simulink model "IEEE_BUS_68_AGC"  (R2025a)
settings: Solver=ode23tb  StartTime=0.0  StopTime=150  FixedStep=Ts  MaxStep=0.0001  RelTol=1e-3
PreLoadFcn:
  | PSSMODEL=1;
  | LPSS=0;
  | WAPSS=0;
  | WAPSS2=0;
  | Ts=50e-5;
InitFcn:
  | PSSMODEL=1;
  | LPSS=0;
  | WAPSS=0;
  | WAPSS2=0;
  | Ts=50e-5;
  | 
  | % Required data to 68 Bus benchmark
  | % clear
  | % clc
  | % Definition for the columns
  | % system base =100 MVA
  | 
  | %% Line data Format (line)
  | % All values are given on the same system base MVA
  | % 1: From bus
  | % 2: To bus
  | % 3: Resistance (pu)
  | % 4: Reactance  (pu)
  | % 5: Charge     (pu)
  | % 6: Transformer Tap Amplitute
  | % 7: base MVA
  | % 8: Nomonal Voltage (KV)
  | 
  | %1   2    3        4       5       6        7      8
  | line=[...
  | 1	54	0	     0.0181	  0	      1.025     100    13.8
  | 2	58	0	     0.025	  0	      1.070     100    13.8
  | 3	62	0	     0.02	  0	      1.070     100    13.8
  | 4	19	0.0007	 0.0142	  0	      1.070     100    13.8
  | 5	20	0.0009	 0.018	  0	      1.009     100    13.8
  | 6	22	0	     0.0143	  0	      1.025     100    13.8
  | 7	23	0.0005	 0.0272	  0	      0         100    13.8
  | 8	25	0.0006	 0.0232	  0	      1.025     100    13.8
  | 9	29	0.0008	 0.0156   0	      1.025     100    13.8
  | 10	31	0	     0.026	  0	      1.04      100    13.8
  | 11	32	0	     0.013	  0	      1.04      100    13.8
  | 12	36	0	     0.0075	  0	      1.04      100    13.8
  | 13	17	0	     0.0033	  0	      1.04      100    13.8
  | 14	41	0	     0.0015	  0	      1         100    13.8
  | 15	42	0	     0.0015	  0	      1         100    13.8
  | 16	18	0	     0.003	  0	      1         100    13.8
  | 17	36	0.0005	 0.0045	  0.32	  0         100    138
  | 17	43	0.0005	 0.0276	  0	      0         100    138
  | 18	42	0.004	 0.06	  2.25    0         100    138
  | 18	49	0.0076	 0.1141	  1.16    0	        100    138
  | 18	50	0.0012	 0.0288	  2.06	  0         100    138
  | 20	19	0.0007	 0.0138	  0       1.06	    100    138
  | 19	68	0.0016	 0.0195	  0.304	  0         100    138
  | 21	22	0.0008	 0.014	  0.2565  0	        100    138
  | 21	68	0.0008	 0.0135	  0.2548  0	        100    138
  | 22	23	0.0006	 0.0096	  0.1846  0	        100    138
  | 23	24	0.0022	 0.035	  0.361	  0         100    138
  | 24	68	0.0003	 0.0059	  0.068	  0         100    138
  | 25	26	0.0032	 0.0323	  0.531	  0         100    138
  | 25	54	0.007	 0.0086	  0.146	  0         100    138
  | 26	27	0.0014	 0.0147	  0.2396  0	        100    138
  | 26	28	0.0043	 0.0474	  0.7802  0	        100    138
  | 26	29	0.0057	 0.0625	  1.029	  0         100    138
  | 27	37	0.0013	 0.0173	  0.3216  0	        100    138
  | 27	53	0.032	 0.32	  0.41	  0         100    138
  | ... (+206 lines)
undefined symbols (not defined in the file or in its folder): D1, Delta
libraries: spsPMUPLLBasedPositiveSequenceLib x90, spsRMSLib x73, spsThreePhaseVIMeasurementLib x69, spsLoadFlowBusLib x69, spsThreePhasePISectionLineLib x64, spsThreePhaseParallelRLCLoadLib x35, spsGenericPowerSystemStabilizerLib x32, spsThreePhaseSeriesRLCLoadLib x21, spsThreePhaseTransformerTwoWindingsLib x21, spsSynchronousMachinepuStandardLib x20, spsExcitationSystemLib x16, spsMultiBandPowerSystemStabilizerLib x16
(part 3 of 8)

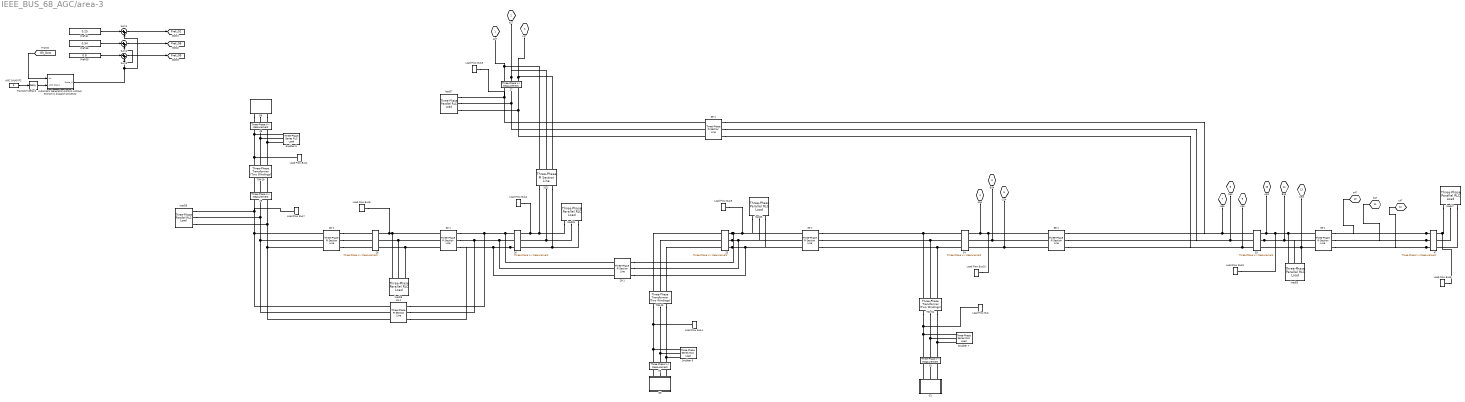
== system IEEE_BUS_68_AGC/area-3 ==
  01 : spsThreePhaseVIMeasurementLib/Three-Phase V-I Measurement  VoltageMeasurement=phase-to-phase  SetLabelV=on  LabelV=Vabc_01  Vpu=off  VpuLL=on  CurrentMeasurement=no  SetLabelI=off  LabelI=Iabc  Ipu=off  Pbase=100e6  Vbase=13.8e3  OutputType=Complex  PhasorSimulation=off  PSBequivalent=0
  08 : spsThreePhaseVIMeasurementLib/Three-Phase V-I Measurement  VoltageMeasurement=phase-to-phase  SetLabelV=on  LabelV=Vabc_08  Vpu=off  VpuLL=on  CurrentMeasurement=no  SetLabelI=off  LabelI=Iabc  Ipu=off  Pbase=100e6  Vbase=13.8e3  OutputType=Complex  PhasorSimulation=off  PSBequivalent=0
  09 : spsThreePhaseVIMeasurementLib/Three-Phase V-I Measurement  VoltageMeasurement=phase-to-phase  SetLabelV=on  LabelV=Vabc_09  Vpu=off  VpuLL=on  CurrentMeasurement=no  SetLabelI=off  LabelI=Iabc  Ipu=off  Pbase=100e6  Vbase=13.8e3  OutputType=Complex  PhasorSimulation=off  PSBequivalent=0
  25 : spsThreePhaseVIMeasurementLib/Three-Phase V-I Measurement  VoltageMeasurement=phase-to-phase  SetLabelV=on  LabelV=Vabc_25  Vpu=off  VpuLL=on  CurrentMeasurement=no  SetLabelI=off  LabelI=Iabc  Ipu=off  Pbase=100e6  Vbase=Bus(25,2)*1e3  OutputType=Complex  PhasorSimulation=off  PSBequivalent=0
  26 : spsThreePhaseVIMeasurementLib/Three-Phase V-I Measurement  VoltageMeasurement=phase-to-phase  SetLabelV=on  LabelV=Vabc_26  Vpu=off  VpuLL=on  CurrentMeasurement=no  SetLabelI=off  LabelI=Iabc  Ipu=off  Pbase=100e6  Vbase=Bus(26,2)*1e3  OutputType=Complex  PhasorSimulation=off  PSBequivalent=0
  27 : spsThreePhaseVIMeasurementLib/Three-Phase V-I Measurement  VoltageMeasurement=phase-to-phase  SetLabelV=on  LabelV=Vabc_27  Vpu=off  VpuLL=on  CurrentMeasurement=no  SetLabelI=off  LabelI=Iabc  Ipu=off  Pbase=100e6  Vbase=Bus(27,2)*1e3  OutputType=Complex  PhasorSimulation=off  PSBequivalent=0
  28 : spsThreePhaseVIMeasurementLib/Three-Phase V-I Measurement  VoltageMeasurement=phase-to-phase  SetLabelV=on  LabelV=Vabc_28  Vpu=off  VpuLL=on  CurrentMeasurement=no  SetLabelI=off  LabelI=Iabc  Ipu=off  Pbase=100e6  Vbase=Bus(28,2)*1e3  OutputType=Complex  PhasorSimulation=off  PSBequivalent=0
  29 : spsThreePhaseVIMeasurementLib/Three-Phase V-I Measurement  VoltageMeasurement=phase-to-phase  SetLabelV=on  LabelV=Vabc_29  Vpu=off  VpuLL=on  CurrentMeasurement=no  SetLabelI=off  LabelI=Iabc  Ipu=off  Pbase=100e6  Vbase=Bus(29,2)*1e3  OutputType=Complex  PhasorSimulation=off  PSBequivalent=0
  29-1 : spsThreePhasePISectionLineLib/Three-Phase PI Section Line  LConnTagsString=a|b|c  RConnTagsString=A|B|C  Length=1  Frequency=60  Resistances=[line(29,3) 3*line(29,3)]  Inductances=[line(29,4) 3*line(29,4)]  Capacitances=[line(29,5) line(29,5)/3]
  30-1 : spsThreePhasePISectionLineLib/Three-Phase PI Section Line  LConnTagsString=a|b|c  RConnTagsString=A|B|C  Length=1  Frequency=60  Resistances=[line(30,3) 3*line(30,3)]  Inductances=[line(30,4) 3*line(30,4)]  Capacitances=[line(30,5) line(30,5)/3]
  31-1 : spsThreePhasePISectionLineLib/Three-Phase PI Section Line  LConnTagsString=a|b|c  RConnTagsString=A|B|C  Length=1  Frequency=60  Resistances=[line(31,3) 3*line(31,3)]  Inductances=[line(31,4) 3*line(31,4)]  Capacitances=[line(31,5) line(31,5)/3]
  32-1 : spsThreePhasePISectionLineLib/Three-Phase PI Section Line  LConnTagsString=a|b|c  RConnTagsString=A|B|C  Length=1  Frequency=60  Resistances=[line(32,3) 3*line(32,3)]  Inductances=[line(32,4) 3*line(32,4)]  Capacitances=[line(32,5) line(32,5)/3]
  33-1 : spsThreePhasePISectionLineLib/Three-Phase PI Section Line  LConnTagsString=a|b|c  RConnTagsString=A|B|C  Length=1  Frequency=60  Resistances=[line(33,3) 3*line(33,3)]  Inductances=[line(33,4) 3*line(33,4)]  Capacitances=[line(33,5) line(33,5)/3]
  35-1 : spsThreePhasePISectionLineLib/Three-Phase PI Section Line  LConnTagsString=a|b|c  RConnTagsString=A|B|C  Length=1  Frequency=60  Resistances=[line(35,3) 3*line(35,3)]  Inductances=[line(35,4) 3*line(35,4)]  Capacitances=[line(35,5) line(35,5)/3]
  36-1 : spsThreePhasePISectionLineLib/Three-Phase PI Section Line  LConnTagsString=a|b|c  RConnTagsString=A|B|C  Length=1  Frequency=60  Resistances=[line(36,3) 3*line(36,3)]  Inductances=[line(36,4) 3*line(36,4)]  Capacitances=[line(36,5) line(36,5)/3]
  47 : spsThreePhaseVIMeasurementLib/Three-Phase V-I Measurement  VoltageMeasurement=phase-to-phase  SetLabelV=on  LabelV=Vabc_47  Vpu=off  VpuLL=on  CurrentMeasurement=no  SetLabelI=off  LabelI=Iabc  Ipu=off  Pbase=100e6  Vbase=Bus(47,2)*1e3  OutputType=Complex  PhasorSimulation=off  PSBequivalent=0
  53 : spsThreePhaseVIMeasurementLib/Three-Phase V-I Measurement  VoltageMeasurement=phase-to-phase  SetLabelV=on  LabelV=Vabc_53  Vpu=off  VpuLL=on  CurrentMeasurement=no  SetLabelI=off  LabelI=Iabc  Ipu=off  Pbase=100e6  Vbase=Bus(53,2)*1e3  OutputType=Complex  PhasorSimulation=off  PSBequivalent=0
  54 : spsThreePhaseVIMeasurementLib/Three-Phase V-I Measurement  VoltageMeasurement=phase-to-phase  SetLabelV=on  LabelV=Vabc_54  Vpu=off  VpuLL=on  CurrentMeasurement=no  SetLabelI=off  LabelI=Iabc  Ipu=off  Pbase=100e6  Vbase=Bus(54,2)*1e3  OutputType=Complex  PhasorSimulation=off  PSBequivalent=0
  63-1 : spsThreePhasePISectionLineLib/Three-Phase PI Section Line  LConnTagsString=a|b|c  RConnTagsString=A|B|C  Length=1  Frequency=60  Resistances=[line(63,3) 3*line(63,3)]  Inductances=[line(63,4) 3*line(63,4)]  Capacitances=[line(63,5) line(63,5)/3]
  66-1 : spsThreePhasePISectionLineLib/Three-Phase PI Section Line  LConnTagsString=a|b|c  RConnTagsString=A|B|C  Length=1  Frequency=60  Resistances=[line(66,3) 3*line(66,3)]  Inductances=[line(66,4) 3*line(66,4)]  Capacitances=[line(66,5) line(66,5)/3]
  AGC ON/OFF2 : Constant
  Automatic Generation Control without economic dispatch process2 : Subsystem
  G1 : Subsystem
  G8 : Subsystem
  G9 : Subsystem
  Load Flow Bus : spsLoadFlowBusLib/Load Flow Bus  LConnTagsString=a  Phases=single  Connectors=on one side  ID=BUS_01  Vbase=13.8e3  Vref=1.045  Vangle=0  VLF=1.045  VLFb=1  VLFc=1  angleLF=-12.3  angleLFb=0  angleLFc=0
  Load Flow Bus1 : spsLoadFlowBusLib/Load Flow Bus  LConnTagsString=a  Phases=single  Connectors=on one side  ID=BUS_09  Vbase=13.8e3  Vref=1.025  Vangle=0  VLF=1.025  VLFb=1  VLFc=1  angleLF=-5.821  angleLFb=0  angleLFc=0
  Load Flow Bus10 : spsLoadFlowBusLib/Load Flow Bus  LConnTagsString=a  Phases=single  Connectors=on one side  ID=BUS_54  Vbase=138e3  Vref=1  Vangle=0  VLF=1.017  VLFb=1  VLFc=1  angleLF=15.31  angleLFb=0  angleLFc=0
  Load Flow Bus2 : spsLoadFlowBusLib/Load Flow Bus  LConnTagsString=a  Phases=single  Connectors=on one side  ID=BUS_26  Vbase=138e3  Vref=1  Vangle=0  VLF=1.035  VLFb=1  VLFc=1  angleLF=15.99  angleLFb=0  angleLFc=0
  Load Flow Bus3 : spsLoadFlowBusLib/Load Flow Bus  LConnTagsString=a  Phases=single  Connectors=on one side  ID=BUS_27  Vbase=138e3  Vref=1  Vangle=0  VLF=1.025  VLFb=1  VLFc=1  angleLF=15.59  angleLFb=0  angleLFc=0
  Load Flow Bus4 : spsLoadFlowBusLib/Load Flow Bus  LConnTagsString=a  Phases=single  Connectors=on one side  ID=BUS_08  Vbase=13.8e3  Vref=1.03  Vangle=0  VLF=1.03  VLFb=1  VLFc=1  angleLF=-6.494  angleLFb=0  angleLFc=0
  Load Flow Bus5 : spsLoadFlowBusLib/Load Flow Bus  LConnTagsString=a  Phases=single  Connectors=on one side  ID=BUS_25  Vbase=138e3  Vref=1  Vangle=0  VLF=1.031  VLFb=1  VLFc=1  angleLF=16.75  angleLFb=0  angleLFc=0
  Load Flow Bus6 : spsLoadFlowBusLib/Load Flow Bus  LConnTagsString=a  Phases=single  Connectors=on one side  ID=BUS_28  Vbase=138e3  Vref=1  Vangle=0  VLF=1.028  VLFb=1  VLFc=1  angleLF=16.68  angleLFb=0  angleLFc=0
  Load Flow Bus7 : spsLoadFlowBusLib/Load Flow Bus  LConnTagsString=a  Phases=single  Connectors=on one side  ID=BUS_29  Vbase=138e3  Vref=1  Vangle=0  VLF=1.02  VLFb=1  VLFc=1  angleLF=17.35  angleLFb=0  angleLFc=0
  Load Flow Bus8 : spsLoadFlowBusLib/Load Flow Bus  LConnTagsString=a  Phases=single  Connectors=on one side  ID=BUS_47  Vbase=138e3  Vref=1  Vangle=0  VLF=1.027  VLFb=1  VLFc=1  angleLF=6.526  angleLFb=0  angleLFc=0
  Load Flow Bus9 : spsLoadFlowBusLib/Load Flow Bus  LConnTagsString=a  Phases=single  Connectors=on one side  ID=BUS_53  Vbase=138e3  Vref=1  Vangle=0  VLF=1.01  VLFb=1  VLFc=1  angleLF=8.812  angleLFb=0  angleLFc=0
  Pref G1 : Constant  Value=0.25
  Pref G8 : Constant  Value=0.54
  Pref G9 : Constant  Value=0.8
  Snubber 5 : spsThreePhaseSeriesRLCLoadLib/Three-Phase Series RLC Load  LConnTagsString=A|B|C  Configuration=Y (grounded)  NominalVoltage=13.8e3  Vabc=[1e3 1e3 1e3]  Vabcp=[1e3 1e3 1e3]  NominalFrequency=60  UnbalancedPower=off  ActivePower=1000000  InductivePower=0  CapacitivePower=10000000  Pabc=[10e3 9e3 11e3]  QLabc=[100 90 110]  QCabc=[100 90 110]  Pabcp=[10e3 9e3 11e3]  QLabcp=[100 90 110]  QCabcp=[100 90 110]  Measurements=None  LoadType=constant Z
  Snubber 6 : spsThreePhaseSeriesRLCLoadLib/Three-Phase Series RLC Load  LConnTagsString=A|B|C  Configuration=Y (grounded)  NominalVoltage=13.8e3  Vabc=[1e3 1e3 1e3]  Vabcp=[1e3 1e3 1e3]  NominalFrequency=60  UnbalancedPower=off  ActivePower=1000000  InductivePower=0  CapacitivePower=10000000  Pabc=[10e3 9e3 11e3]  QLabc=[100 90 110]  QCabc=[100 90 110]  Pabcp=[10e3 9e3 11e3]  QLabcp=[100 90 110]  QCabcp=[100 90 110]  Measurements=None  LoadType=constant Z
  Snubber 7 : spsThreePhaseSeriesRLCLoadLib/Three-Phase Series RLC Load  LConnTagsString=A|B|C  Configuration=Y (grounded)  NominalVoltage=13.8e3  Vabc=[1e3 1e3 1e3]  Vabcp=[1e3 1e3 1e3]  NominalFrequency=60  UnbalancedPower=off  ActivePower=1000000  InductivePower=0  CapacitivePower=10000000  Pabc=[10e3 9e3 11e3]  QLabc=[100 90 110]  QCabc=[100 90 110]  Pabcp=[10e3 9e3 11e3]  QLabcp=[100 90 110]  QCabcp=[100 90 110]  Measurements=None  LoadType=constant Z
  Sum1 : Sum  Inputs=|++
  Sum4 : Sum  Inputs=|++
  Sum5 : Sum  Inputs=|++
  T01-54 : spsThreePhaseTransformerTwoWindingsLib/Three-Phase Transformer (Two Windings)  Winding1Connection=Delta (D1)  Winding2Connection=Yg  CoreType=Three single-phase transformers  SetSaturation=off  Hysteresis=off  DataFile='hysteresis'  SetInitialFlux=off  Measurements=None  UNITS=pu  NominalPower=[ 100e6 , 60 ]  Winding1=[ 13.8e3 , 0.0002 , 0 ]  Winding2=[ 138e3 , 0.0002, 0.0181]  Rm=500  Lm=500  L0=0.5  Saturation=[ 0,0 ; 0.0024,1.2 ; 1.0,1.52 ]  InitialFluxes=[ 0.8 , -0.8 , 0.7 ]  BreakLoop=off  DiscreteSolver=Trapezoidal robust  DataType=off  TransfoNumber=1
  T08-25 : spsThreePhaseTransformerTwoWindingsLib/Three-Phase Transformer (Two Windings)  Winding1Connection=Delta (D1)  Winding2Connection=Yg  CoreType=Three single-phase transformers  SetSaturation=off  Hysteresis=off  DataFile='hysteresis'  SetInitialFlux=off  Measurements=None  UNITS=pu  NominalPower=[ 100e6 , 60 ]  Winding1=[ 13.8e3 , 0.0003 , 0 ]  Winding2=[ 138e3 , 0.0003, 0.0232]  Rm=500  Lm=500  L0=0.5  Saturation=[ 0,0 ; 0.0024,1.2 ; 1.0,1.52 ]  InitialFluxes=[ 0.8 , -0.8 , 0.7 ]  BreakLoop=off  DiscreteSolver=Trapezoidal robust  DataType=off  TransfoNumber=1
  T09-29 : spsThreePhaseTransformerTwoWindingsLib/Three-Phase Transformer (Two Windings)  Winding1Connection=Delta (D1)  Winding2Connection=Yg  CoreType=Three single-phase transformers  SetSaturation=off  Hysteresis=off  DataFile='hysteresis'  SetInitialFlux=off  Measurements=None  UNITS=pu  NominalPower=[ 100e6 , 60 ]  Winding1=[ 13.8e3 , 0.0004 , 0 ]  Winding2=[ 138e3 , 0.0004 , 0.0156]  Rm=500  Lm=500  L0=0.5  Saturation=[ 0,0 ; 0.0024,1.2 ; 1.0,1.52 ]  InitialFluxes=[ 0.8 , -0.8 , 0.7 ]  BreakLoop=off  DiscreteSolver=Trapezoidal robust  DataType=off  TransfoNumber=1
  Transport Delay2 : TransportDelay  DelayTime=20
  load25 : spsThreePhaseParallelRLCLoadLib/Three-Phase Parallel RLC Load  LConnTagsString=A|B|C  Configuration=Y (grounded)  NominalVoltage=(138000)*1.03119  Vabc=[1e3 1e3 1e3]  Vabcp=[1e3 1e3 1e3]  NominalFrequency=60  UnbalancedPower=off  ActivePower=224000000  InductivePower=47000000  CapacitivePower=0  Pabc=[10e3 9e3 11e3]  QLabc=[100 90 110]  QCabc=[100 90 110]  Pabcp=[10e3 9e3 11e3]  QLabcp=[100 90 110]  QCabcp=[100 90 110]  Measurements=None  LoadType=constant PQ
  load26 : spsThreePhaseParallelRLCLoadLib/Three-Phase Parallel RLC Load  LConnTagsString=A|B|C  Configuration=Y (grounded)  NominalVoltage=(138000)*1.03517  Vabc=[1e3 1e3 1e3]  Vabcp=[1e3 1e3 1e3]  NominalFrequency=60  UnbalancedPower=off  ActivePower=50000000  InductivePower=7000000  CapacitivePower=0  Pabc=[10e3 9e3 11e3]  QLabc=[100 90 110]  QCabc=[100 90 110]  Pabcp=[10e3 9e3 11e3]  QLabcp=[100 90 110]  QCabcp=[100 90 110]  Measurements=None  LoadType=constant PQ
  load27 : spsThreePhaseParallelRLCLoadLib/Three-Phase Parallel RLC Load  LConnTagsString=A|B|C  Configuration=Y (grounded)  NominalVoltage=(138000)*1.02502  Vabc=[1e3 1e3 1e3]  Vabcp=[1e3 1e3 1e3]  NominalFrequency=60  UnbalancedPower=off  ActivePower=130000000  InductivePower=20000000  CapacitivePower=0  Pabc=[10e3 9e3 11e3]  QLabc=[100 90 110]  QCabc=[100 90 110]  Pabcp=[10e3 9e3 11e3]  QLabcp=[100 90 110]  QCabcp=[100 90 110]  Measurements=None  LoadType=constant PQ
  load28 : spsThreePhaseParallelRLCLoadLib/Three-Phase Parallel RLC Load  LConnTagsString=A|B|C  Configuration=Y (grounded)  NominalVoltage=(138000)*1.02808  Vabc=[1e3 1e3 1e3]  Vabcp=[1e3 1e3 1e3]  NominalFrequency=60  UnbalancedPower=off  ActivePower=50000000  InductivePower=7000000  CapacitivePower=0  Pabc=[10e3 9e3 11e3]  QLabc=[100 90 110]  QCabc=[100 90 110]  Pabcp=[10e3 9e3 11e3]  QLabcp=[100 90 110]  QCabcp=[100 90 110]  Measurements=None  LoadType=constant PQ
  load29 : spsThreePhaseParallelRLCLoadLib/Three-Phase Parallel RLC Load  LConnTagsString=A|B|C  Configuration=Y (grounded)  NominalVoltage=(138000)*1.01962  Vabc=[1e3 1e3 1e3]  Vabcp=[1e3 1e3 1e3]  NominalFrequency=60  UnbalancedPower=off  ActivePower=680000000  InductivePower=106000000  CapacitivePower=0  Pabc=[10e3 9e3 11e3]  QLabc=[100 90 110]  QCabc=[100 90 110]  Pabcp=[10e3 9e3 11e3]  QLabcp=[100 90 110]  QCabcp=[100 90 110]  Measurements=None  LoadType=constant PQ
  load47 : spsThreePhaseParallelRLCLoadLib/Three-Phase Parallel RLC Load  LConnTagsString=A|B|C  Configuration=Y (grounded)  NominalVoltage=(138000)*1.02686  Vabc=[1e3 1e3 1e3]  Vabcp=[1e3 1e3 1e3]  NominalFrequency=60  UnbalancedPower=off  ActivePower=203000000  InductivePower=33000000  CapacitivePower=0  Pabc=[10e3 9e3 11e3]  QLabc=[100 90 110]  QCabc=[100 90 110]  Pabcp=[10e3 9e3 11e3]  QLabcp=[100 90 110]  QCabcp=[100 90 110]  Measurements=None  LoadType=constant PQ
  load53 : spsThreePhaseParallelRLCLoadLib/Three-Phase Parallel RLC Load  LConnTagsString=A|B|C  Configuration=Y (grounded)  NominalVoltage=(138000)*1.01027  Vabc=[1e3 1e3 1e3]  Vabcp=[1e3 1e3 1e3]  NominalFrequency=60  UnbalancedPower=off  ActivePower=253000000  InductivePower=119000000  CapacitivePower=0  Pabc=[10e3 9e3 11e3]  QLabc=[100 90 110]  QCabc=[100 90 110]  Pabcp=[10e3 9e3 11e3]  QLabcp=[100 90 110]  QCabcp=[100 90 110]  Measurements=None  LoadType=constant PQ
  a27 : PMIOPort  Tag=PMCPort  Side=Right
  b27 : PMIOPort  Tag=PMCPort  Port=2  Side=Right
  c27 : PMIOPort  Tag=PMCPort  Port=3  Side=Right
  A54 : PMIOPort  Tag=PMCPort  Port=4  Side=Right
  B54 : PMIOPort  Tag=PMCPort  Port=5  Side=Right
  C54 : PMIOPort  Tag=PMCPort  Port=6  Side=Right
  a53 : PMIOPort  Tag=PMCPort  Port=7  Side=Right
  b53 : PMIOPort  Tag=PMCPort  Port=8  Side=Right
  c53 : PMIOPort  Tag=PMCPort  Port=9  Side=Right
  a47 : PMIOPort  Tag=PMCPort  Port=10  Side=Right
  b47 : PMIOPort  Tag=PMCPort  Port=11  Side=Right
  c47 : PMIOPort  Tag=PMCPort  Port=12  Side=Right
  C53 : PMIOPort  Tag=PMCPort  Port=13  Side=Right
  B53 : PMIOPort  Tag=PMCPort  Port=14  Side=Right
  A53 : PMIOPort  Tag=PMCPort  Port=15  Side=Right
  tag scope: Pref_G1=global, Pref_G8=global, Pref_G9=global
  wires:
  Pref G9/1 -> Sum5/1
  Transport Delay2/1 -> Automatic Generation Control without economic dispatch process2/2(AGC Status)
  AGC ON/OFF2/1 -> Transport Delay2/1
  [G9_Goto] -> Automatic Generation Control without economic dispatch process2/1(dw)
  Sum4/1 -> [Pref_G8]
  Pref G1/1 -> Sum1/1
  Pref G8/1 -> Sum4/1
  Sum5/1 -> [Pref_G9]
  Sum1/1 -> [Pref_G1]
  Automatic Generation Control without economic dispatch process2/1(Delta_P) -> Sum1/2, Sum4/2, Sum5/2
  connections:
  T09-29/LConn1 -- Snubber 5/LConn1 -- 09/LConn1 -- Load Flow Bus1/LConn1
  G9/LConn1 -- 09/RConn1
  G9/LConn2 -- 09/RConn2
  G9/LConn3 -- 09/RConn3
  T09-29/LConn3 -- Snubber 5/LConn3 -- 09/LConn3
  T09-29/LConn2 -- Snubber 5/LConn2 -- 09/LConn2
  29/RConn1 -- T09-29/RConn1
  29/RConn2 -- T09-29/RConn2
  29/RConn3 -- T09-29/RConn3
  33-1/RConn1 -- load29/LConn1 -- 29/LConn1 -- Load Flow Bus7/LConn1 -- 36-1/RConn1
  36-1/RConn2 -- load29/LConn2 -- 29/LConn2 -- 33-1/RConn2
  36-1/RConn3 -- load29/LConn3 -- 29/LConn3 -- 33-1/RConn3
  36-1/LConn1 -- 28/RConn1
  36-1/LConn2 -- 28/RConn2
  36-1/LConn3 -- 28/RConn3
  32-1/RConn1 -- load28/LConn1 -- Load Flow Bus6/LConn1 -- 28/LConn1
  32-1/RConn2 -- load28/LConn2 -- 28/LConn2
  32-1/RConn3 -- load28/LConn3 -- 28/LConn3
  32-1/LConn1 -- 33-1/LConn1 -- 26/RConn1 -- 29-1/LConn1
  32-1/LConn2 -- 33-1/LConn2 -- 26/RConn2 -- 29-1/LConn2
  26/RConn3 -- 32-1/LConn3 -- 33-1/LConn3 -- 29-1/LConn3
  load27/LConn1 -- 35-1/RConn1 -- Load Flow Bus3/LConn1 -- 27/LConn1
  load27/LConn2 -- 27/LConn2 -- 35-1/RConn2
  load27/LConn3 -- 27/LConn3 -- 35-1/RConn3
  T08-25/RConn1 -- 25/RConn1
  T08-25/RConn2 -- 25/RConn2
  T08-25/RConn3 -- 25/RConn3
  load26/LConn1 -- 31-1/RConn1 -- Load Flow Bus2/LConn1 -- 26/LConn1
  load26/LConn2 -- 31-1/RConn2 -- 26/LConn2
  load26/LConn3 -- 31-1/RConn3 -- 26/LConn3
  G8/LConn1 -- 08/RConn1
  G8/LConn2 -- 08/RConn2
  G8/LConn3 -- 08/RConn3
  T08-25/LConn1 -- Load Flow Bus4/LConn1 -- Snubber 6/LConn1 -- 08/LConn1
  T08-25/LConn2 -- Snubber 6/LConn2 -- 08/LConn2
  T08-25/LConn3 -- Snubber 6/LConn3 -- 08/LConn3
  25/LConn1 -- Load Flow Bus5/LConn1 -- 30-1/RConn1 -- load25/LConn1 -- 29-1/RConn1
  25/LConn2 -- 30-1/RConn2 -- load25/LConn2 -- 29-1/RConn2
  25/LConn3 -- 30-1/RConn3 -- load25/LConn3 -- 29-1/RConn3
  30-1/LConn1 -- T01-54/RConn1 -- 54/RConn1
  30-1/LConn2 -- T01-54/RConn2 -- 54/RConn2
  30-1/LConn3 -- T01-54/RConn3 -- 54/RConn3
  T01-54/LConn1 -- 01/LConn1 -- Snubber 7/LConn1 -- Load Flow Bus/LConn1
  T01-54/LConn2 -- 01/LConn2 -- Snubber 7/LConn2
  T01-54/LConn3 -- 01/LConn3 -- Snubber 7/LConn3
  G1/LConn1 -- 01/RConn1
  G1/LConn2 -- 01/RConn2
  G1/LConn3 -- 01/RConn3
  66-1/RConn1 -- Load Flow Bus10/LConn1 -- 54/LConn1 -- A54/RConn1
  66-1/RConn2 -- 54/LConn2 -- B54/RConn1
  66-1/RConn3 -- C54/RConn1 -- 54/LConn3
  a53/RConn1 -- 53/RConn1 -- 66-1/LConn1 -- 35-1/LConn1
  b53/RConn1 -- 53/RConn2 -- 66-1/LConn2 -- 35-1/LConn2
  c53/RConn1 -- 53/RConn3 -- 66-1/LConn3 -- 35-1/LConn3
  63-1/RConn1 -- load53/LConn1 -- Load Flow Bus9/LConn1 -- 53/LConn1 -- A53/RConn1
  53/LConn2 -- load53/LConn2 -- 63-1/RConn2 -- B53/RConn1
  63-1/RConn3 -- 53/LConn3 -- load53/LConn3 -- C53/RConn1
  47/RConn1 -- 63-1/LConn1 -- a47/RConn1
  47/RConn2 -- 63-1/LConn2 -- b47/RConn1
  47/RConn3 -- 63-1/LConn3 -- c47/RConn1
  31-1/LConn1 -- a27/RConn1 -- 27/RConn1
  27/RConn2 -- b27/RConn1 -- 31-1/LConn2
  27/RConn3 -- c27/RConn1 -- 31-1/LConn3
  load47/LConn1 -- Load Flow Bus8/LConn1 -- 47/LConn1
  load47/LConn2 -- 47/LConn2
  load47/LConn3 -- 47/LConn3
